simulink model "AdaptiveCruiseRoughIn2023a"  (R2025b)
settings: Solver=ode3  StartTime=0.0  StopTime=10  FixedStep=0.01  RelTol=1e-3  EnableMultiTasking=on
settings Model: Creator=zmxie  LastModifiedBy=grantdahl
settings SolverCC: AlgebraicLoopSolver=TrustRegion
settings DataIOCC: LimitDataPoints=on  SaveFormat=Array  SignalLoggingSaveFormat=ModelDataLogs  ReturnWorkspaceOutputs=off
settings OptimizationCC: BooleanDataType=off
settings DebuggingCC: SaveWithParameterizedLinksMsg=none  UnderspecifiedInitializationDetection=Classic  MergeDetectMultiDrivingBlocksExec=none  SignalResolutionControl=TryResolveAllWithWarning  MultiTaskDSMMsg=warning  MultiTaskCondExecSysMsg=none  UnconnectedInputMsg=warning  UnconnectedOutputMsg=warning  UnconnectedLineMsg=warning  ArithmeticOperatorsInVariantConditions=warning
settings HardwareCC: TargetUnknown=on
settings ModelReferenceCC: EnableRefExpFcnMdlSchedulingChecks=on  PropagateSignalLabelsOutOfModel=off
settings SFSimCC: SimUseLocalCustomCode=off  CustomCodeUndefinedFunction=UseInterfaceOnly
settings RTWCC: RTWUseLocalCustomCode=off  GPUComputeCapability=3.5
settings CodeAppCC: StateflowObjectComments=on
settings GRTTargetCC: TargetLangStandard=C89/C90 (ANSI)  CombineOutputUpdateFcns=off  GRTInterface=on
settings ConfigComp: CovMetricSettings=dw  CovSaveCumulativeToWorkspaceVar=on  CovSaveSingleToWorkspaceVar=on  CovExternalEMLEnable=off

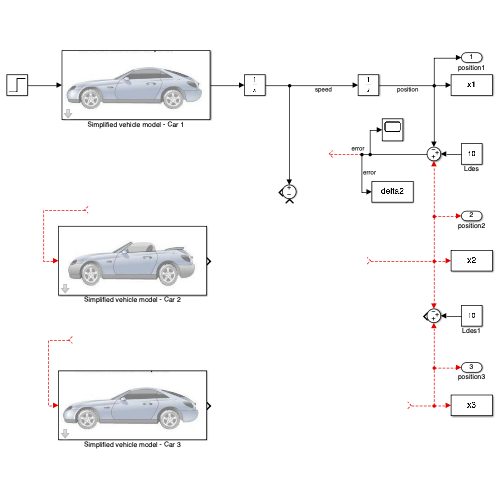
[thumbnail: Simulink's stored preview of the top-level diagram]
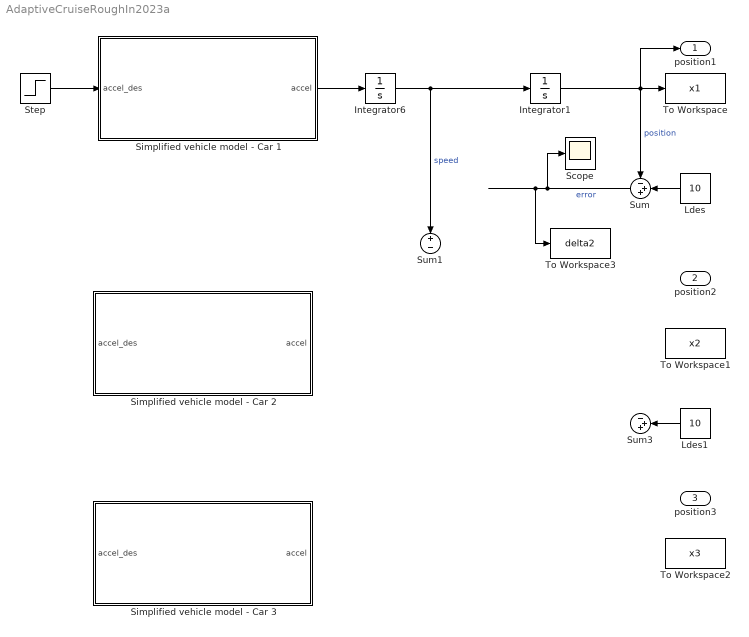
== system AdaptiveCruiseRoughIn2023a ==
  Integrator1 : Integrator
  Integrator6 : Integrator  InitialCondition=30
  Ldes : Constant  Value=10
  Ldes1 : Constant  Value=10
  Scope : Scope
      settings: ActiveDisplayYMinimum=-2.1972  ActiveDisplayYMaximum=2.4664
  Simplified vehicle model - Car 1 : Subsystem  mask(Vehicle model){}
      mask help: Vehicle model
      mask Display: image('sedan.png');
  Simplified vehicle model - Car 2 : Subsystem  mask(Vehicle model){}
      mask help: Vehicle model
      mask Display: image('convertible.png');
  Simplified vehicle model - Car 3 : Subsystem  mask(Vehicle model){}
      mask help: Vehicle model
      mask Display: image('sedan.png');
  Step : Step  SampleTime=0
  Sum : Sum  Inputs=-++
  Sum1 : Sum  Inputs=+-
  Sum3 : Sum  Inputs=-++
  To Workspace : ToWorkspace  VariableName=x1  SaveFormat=Timeseries  SampleTime=-1
  To Workspace1 : ToWorkspace  VariableName=x2  SaveFormat=Timeseries  SampleTime=-1
  To Workspace2 : ToWorkspace  VariableName=x3  SaveFormat=Timeseries  SampleTime=-1
  To Workspace3 : ToWorkspace  VariableName=delta2  SaveFormat=Timeseries  SampleTime=-1
  position1 : Outport
  position2 : Outport  Port=2
  position3 : Outport  Port=3
  wires:
  Step/1 -> Simplified vehicle model - Car 1/1(accel_des)
  Integrator1/1 -> position1/1, To Workspace/1, Sum/1  "position"
  Ldes/1 -> Sum/2
  ? -> Sum3/1, To Workspace1/1, position2/1, Sum/3
  ? -> Simplified vehicle model - Car 2/1(accel_des)
  Sum/1 -> Scope/1, To Workspace3/1  "error"
  Integrator6/1 -> Sum1/1, Integrator1/1  "speed"
  Simplified vehicle model - Car 1/1(accel) -> Integrator6/1
  ? -> Simplified vehicle model - Car 3/1(accel_des)
  Ldes1/1 -> Sum3/2
  ? -> To Workspace2/1, position3/1, Sum3/3

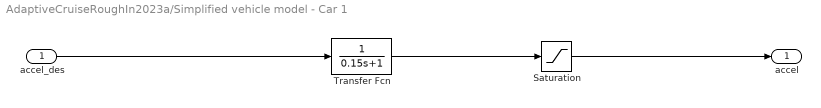
== system AdaptiveCruiseRoughIn2023a/Simplified vehicle model - Car 1 ==
  accel_des : Inport
  Saturation : Saturate  UpperLimit=2.5  LowerLimit=-5
  Transfer Fcn : TransferFcn  Denominator=[0.15 1]
  accel : Outport
  wires:
  Saturation/1 -> accel/1
  Transfer Fcn/1 -> Saturation/1
  accel_des/1 -> Transfer Fcn/1

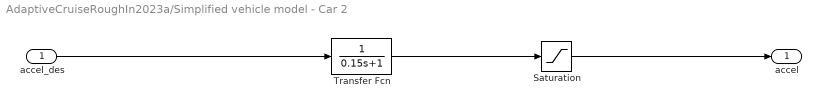
== system AdaptiveCruiseRoughIn2023a/Simplified vehicle model - Car 2 ==
  accel_des : Inport
  Saturation : Saturate  UpperLimit=2.5  LowerLimit=-5
  Transfer Fcn : TransferFcn  Denominator=[0.15 1]
  accel : Outport
  wires:
  Saturation/1 -> accel/1
  Transfer Fcn/1 -> Saturation/1
  accel_des/1 -> Transfer Fcn/1

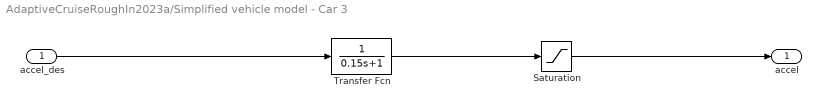
== system AdaptiveCruiseRoughIn2023a/Simplified vehicle model - Car 3 ==
  accel_des : Inport
  Saturation : Saturate  UpperLimit=2.5  LowerLimit=-5
  Transfer Fcn : TransferFcn  Denominator=[0.15 1]
  accel : Outport
  wires:
  Saturation/1 -> accel/1
  Transfer Fcn/1 -> Saturation/1
  accel_des/1 -> Transfer Fcn/1
